simulink model "Dc_motor_simulink_modeling"  (R2020a)
settings: Solver=VariableStepAuto  StartTime=0.0  StopTime=5  RelTol=1e-3
libraries: simulink x1
settings Model: Creator=hp  LastModifiedBy=hp

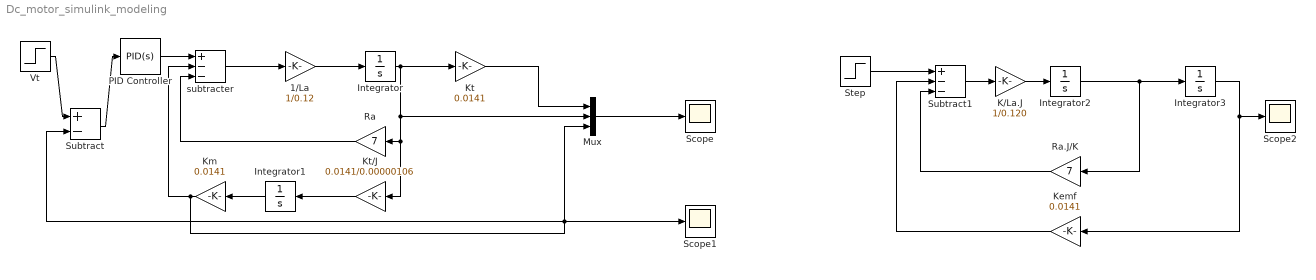
== system Dc_motor_simulink_modeling ==
  1/La : Gain  Gain=1/0.12
  Integrator{,1..3} (4 alike) : Integrator
  K/La.J : Gain  Gain=1/0.120
  Kemf : Gain  Gain=0.0141
  Km : Gain  Gain=0.0141
  Kt : Gain  Gain=0.0141
  Kt/J : Gain  Gain=0.0141/0.00000106
  Mux : Mux  Inputs=3
  PID Controller : simulink/Continuous/PID Controller  Controller=PID  Form=Parallel  TimeDomain=Continuous-time  UseExternalTs=off  SampleTime=-1  IntegratorMethod=Forward Euler  FilterMethod=Forward Euler  ControllerParametersSource=internal  P=1  I=1  D=0  UseFilter=on  N=100  TunerSelectOption=Transfer Function Based (PID Tuner App)  InitialConditionSource=internal  InitialConditionForIntegrator=0  InitialConditionForFilter=0  DifferentiatorICPrevScaledInput=0  ExternalReset=none  TrackingMode=off  Kt=1  LimitOutput=off  UpperSaturationLimit=inf  LowerSaturationLimit=-inf  LinearizeAsGain=on  AntiWindupMode=none  Kb=1  POutMin=[]  POutMax=[]  IOutMin=[]  IOutMax=[]  DOutMin=[]  DOutMax=[]  NOutMin=[]  NOutMax=[]  SumOutMin=[]  SumOutMax=[]  SaturationOutMin=[]  SaturationOutMax=[]  PParamMin=[]  PParamMax=[]  IParamMin=[]  IParamMax=[]  DParamMin=[]  DParamMax=[]  NParamMin=[]  NParamMax=[]  KbParamMin=[]  KbParamMax=[]  KtParamMin=[]  KtParamMax=[]  KbOutMin=[]  KbOutMax=[]  KtOutMin=[]  KtOutMax=[]  IntegratorOutMin=[]  IntegratorOutMax=[]  FilterOutMin=[]  FilterOutMax=[]  SumI1OutMin=[]  SumI1OutMax=[]  SumI2OutMin=[]  SumI2OutMax=[]  SumI3OutMin=[]  SumI3OutMax=[]  SumI4OutMin=[]  SumI4OutMax=[]  SumDOutMin=[]  SumDOutMax=[]  DifferentiatorOutMin=[]  DifferentiatorOutMax=[]  FilterDiffOutCoefMin=[]  FilterDiffOutCoefMax=[]  ReciprocalOutMin=[]  ReciprocalOutMax=[]  SumDenOutMin=[]  SumDenOutMax=[]  SumNumOutMin=[]  SumNumOutMax=[]  DivideOutMin=[]  DivideOutMax=[]  UdiffTsProdOutMin=[]  UdiffTsProdOutMax=[]  NTsProdOutMin=[]  NTsProdOutMax=[]  UintegralTsProdOutMin=[]  UintegralTsProdOutMax=[]  UngainTsProdOutMin=[]  UngainTsProdOutMax=[]  IntegratorContinuousStateAttributes=''  IntegratorStateMustResolveToSignalObject=off  IntegratorRTWStateStorageClass=Auto  FilterContinuousStateAttributes=''  FilterStateMustResolveToSignalObject=off  FilterRTWStateStorageClass=Auto  ParallelPVariant=InternalParameters  IdealPVariant=Disabled  IVariant=InternalParameters  DVariant=InternalParameters  IntegratorVariant=Continuous  SatVariant=Disabled  AWVariant=Passthrough  PCopyVariant=Disabled  TRVariant=Disabled  FdbkBlocksVariant=Forward  IdealPFdbkVariant=Disabled  SatFdbkVariant=Disabled  DerivativeFilterVariant=ContFilter  NVariant=InternalParameters  NCopyVariant=Disabled  FilterICVariant=InternalICsFilter  IntegratorICVariant=InternalICs  ExternalResetVariant=Disabled  TRSumVariant=Passthrough  SumFdbkVariant=Disabled  SumVariant=Sum_PID  TsampFilterVariant=InternalTs  TsampNgainVariant=Passthrough  TsampIntegralVariant=Passthrough
  Ra : Gain  Gain=7
  Ra.J/K : Gain  Gain=7
  Scope : Scope
  Scope1 : Scope
  Scope2 : Scope
  Step : Step  Time=6  SampleTime=0
  Subtract : Sum  Inputs=+-
  Subtract1 : Sum  Inputs=+--
  Vt : Step  Time=5  SampleTime=0
  subtracter : Sum  Inputs=+--
  wires:
  subtracter/1 -> 1/La/1
  1/La/1 -> Integrator/1
  Integrator/1 -> Mux/2, Kt/J/1, Ra/1, Kt/1
  Ra/1 -> subtracter/3
  Kt/J/1 -> Integrator1/1
  Integrator1/1 -> Km/1
  Km/1 -> Subtract/2, Scope1/1, Mux/3, subtracter/2
  Kt/1 -> Mux/1
  Mux/1 -> Scope/1
  Step/1 -> Subtract1/1
  Integrator2/1 -> Ra.J/K/1, Integrator3/1
  Ra.J/K/1 -> Subtract1/3
  Integrator3/1 -> Kemf/1, Scope2/1
  Kemf/1 -> Subtract1/2
  Subtract1/1 -> K/La.J/1
  K/La.J/1 -> Integrator2/1
  PID Controller/1 -> subtracter/1
  Vt/1 -> Subtract/1
  Subtract/1 -> PID Controller/1
